simulink model "kay1024_freq_16ch_test"  (R2021b)
settings: Solver=VariableStepAuto  StartTime=0.0  StopTime=10.0  RelTol=1e-3
undefined symbols (not defined in the file): i
libraries: hdlBasic x1194, dspsrcs4 x16, vmcUtilities x1
(part 9 of 14)

== system kay1024_freq_16ch_test/Subsystem/Subsystem16/Subsystem2/CORDIC ATAN/CORDIC Fine Angle PE/CORDIC PE11 ==
  note: X = x - y if y < 0, otherwise
      |    = x + y
      | Y = y + x if y < 0, otherwise
      |    = y - x
      | Z = z - atan(1/2^i) if y < 0, otherwise
      |    = z + atan(1/2^i)
  x : Inport
  y : Inport  Port=2
  z : Inport  Port=3
  AddSub : hdlBasic/AddSub  mode=Addition or Subtraction  use_carryin=off  use_carryout=off  en=off  latency=pipeline  precision=User Defined  arith_type="Signed  (2's comp)"  n_bits=pe_nbits  bin_pt=pe_binpt  quantization=Truncate  overflow=Wrap  use_behavioral_HDL=on  hw_selection=Fabric  pipelined=off  use_rpm=off  XmcBlockStatus=1  maskContainerNames=tabcontainer1  block_type=addsub  block_config=sysgen:Addsub_config
  AddSub1 : hdlBasic/AddSub  mode=Addition or Subtraction  use_carryin=off  use_carryout=off  en=off  latency=pipeline  precision=User Defined  arith_type="Signed  (2's comp)"  n_bits=pe_nbits  bin_pt=pe_binpt  quantization=Truncate  overflow=Wrap  use_behavioral_HDL=on  hw_selection=Fabric  pipelined=off  use_rpm=off  XmcBlockStatus=1  maskContainerNames=tabcontainer1  block_type=addsub  block_config=sysgen:Addsub_config
  AddSub2 : hdlBasic/AddSub  mode=Addition or Subtraction  use_carryin=off  use_carryout=off  en=off  latency=pipeline  precision=User Defined  arith_type="Signed  (2's comp)"  n_bits=pe_nbits  bin_pt=pe_binpt  quantization=Truncate  overflow=Wrap  use_behavioral_HDL=on  hw_selection=Fabric  pipelined=off  use_rpm=off  XmcBlockStatus=1  maskContainerNames=tabcontainer1  block_type=addsub  block_config=sysgen:Addsub_config
  Constant : hdlBasic/Constant  const=epsilon_k  gui_display_data_type=Fixed-point  arith_type=Signed (2's comp)  n_bits=pe_nbits  bin_pt=pe_binpt  preci_type=Single  exp_width=8  frac_width=24  explicit_period=off  period=1  XmcBlockStatus=1  maskContainerNames=tabcontainer1  block_type=constant  block_config=sysgen:Constant_config
  Inverter : hdlBasic/Inverter  en=off  latency=0  XmcBlockStatus=1  maskContainerNames=group2  block_type=inv  block_config=sysgen:Inverter_config
  Shift : hdlBasic/Shift  shift_dir=Right  shift_bits=ii  en=off  latency=0  precision=User Defined  arith_type="Signed  (2's comp)"  n_bits=pe_nbits  bin_pt=pe_binpt  quantization=Truncate  overflow=Wrap  XmcBlockStatus=1  maskContainerNames=group2  block_type=shift  block_config=sysgen:Shift_config
  Shift1 : hdlBasic/Shift  shift_dir=Right  shift_bits=ii  en=off  latency=0  precision=User Defined  arith_type="Signed  (2's comp)"  n_bits=pe_nbits  bin_pt=pe_binpt  quantization=Truncate  overflow=Wrap  XmcBlockStatus=1  maskContainerNames=group2  block_type=shift  block_config=sysgen:Shift_config
  Slice : hdlBasic/Slice  nbits=1  boolean_output=on  mode=Upper Bit Location + Width  bit1=0  base1=MSB of Input  bit0=0  base0=LSB of Input  XmcBlockStatus=1  maskContainerNames=group1  block_type=slice  block_config=sysgen:Slice_config
  X : Outport
  Y : Outport  Port=2
  Z : Outport  Port=3
  wires:
  Slice/1 -> AddSub/3, AddSub2/3, Inverter/1
  Shift1/1 -> AddSub/2
  Shift/1 -> AddSub1/2
  Inverter/1 -> AddSub1/3
  Constant/1 -> AddSub2/2
  AddSub2/1 -> Z/1
  AddSub1/1 -> Y/1
  z/1 -> AddSub2/1
  AddSub/1 -> X/1
  y/1 -> Slice/1, Shift1/1, AddSub1/1
  x/1 -> Shift/1, AddSub/1

== system kay1024_freq_16ch_test/Subsystem/Subsystem16/Subsystem2/CORDIC ATAN/CORDIC Fine Angle PE/CORDIC PE12 ==
  note: X = x - y if y < 0, otherwise
      |    = x + y
      | Y = y + x if y < 0, otherwise
      |    = y - x
      | Z = z - atan(1/2^i) if y < 0, otherwise
      |    = z + atan(1/2^i)
  x : Inport
  y : Inport  Port=2
  z : Inport  Port=3
  AddSub : hdlBasic/AddSub  mode=Addition or Subtraction  use_carryin=off  use_carryout=off  en=off  latency=pipeline  precision=User Defined  arith_type="Signed  (2's comp)"  n_bits=pe_nbits  bin_pt=pe_binpt  quantization=Truncate  overflow=Wrap  use_behavioral_HDL=on  hw_selection=Fabric  pipelined=off  use_rpm=off  XmcBlockStatus=1  maskContainerNames=tabcontainer1  block_type=addsub  block_config=sysgen:Addsub_config
  AddSub1 : hdlBasic/AddSub  mode=Addition or Subtraction  use_carryin=off  use_carryout=off  en=off  latency=pipeline  precision=User Defined  arith_type="Signed  (2's comp)"  n_bits=pe_nbits  bin_pt=pe_binpt  quantization=Truncate  overflow=Wrap  use_behavioral_HDL=on  hw_selection=Fabric  pipelined=off  use_rpm=off  XmcBlockStatus=1  maskContainerNames=tabcontainer1  block_type=addsub  block_config=sysgen:Addsub_config
  AddSub2 : hdlBasic/AddSub  mode=Addition or Subtraction  use_carryin=off  use_carryout=off  en=off  latency=pipeline  precision=User Defined  arith_type="Signed  (2's comp)"  n_bits=pe_nbits  bin_pt=pe_binpt  quantization=Truncate  overflow=Wrap  use_behavioral_HDL=on  hw_selection=Fabric  pipelined=off  use_rpm=off  XmcBlockStatus=1  maskContainerNames=tabcontainer1  block_type=addsub  block_config=sysgen:Addsub_config
  Constant : hdlBasic/Constant  const=epsilon_k  gui_display_data_type=Fixed-point  arith_type=Signed (2's comp)  n_bits=pe_nbits  bin_pt=pe_binpt  preci_type=Single  exp_width=8  frac_width=24  explicit_period=off  period=1  XmcBlockStatus=1  maskContainerNames=tabcontainer1  block_type=constant  block_config=sysgen:Constant_config
  Inverter : hdlBasic/Inverter  en=off  latency=0  XmcBlockStatus=1  maskContainerNames=group2  block_type=inv  block_config=sysgen:Inverter_config
  Shift : hdlBasic/Shift  shift_dir=Right  shift_bits=ii  en=off  latency=0  precision=User Defined  arith_type="Signed  (2's comp)"  n_bits=pe_nbits  bin_pt=pe_binpt  quantization=Truncate  overflow=Wrap  XmcBlockStatus=1  maskContainerNames=group2  block_type=shift  block_config=sysgen:Shift_config
  Shift1 : hdlBasic/Shift  shift_dir=Right  shift_bits=ii  en=off  latency=0  precision=User Defined  arith_type="Signed  (2's comp)"  n_bits=pe_nbits  bin_pt=pe_binpt  quantization=Truncate  overflow=Wrap  XmcBlockStatus=1  maskContainerNames=group2  block_type=shift  block_config=sysgen:Shift_config
  Slice : hdlBasic/Slice  nbits=1  boolean_output=on  mode=Upper Bit Location + Width  bit1=0  base1=MSB of Input  bit0=0  base0=LSB of Input  XmcBlockStatus=1  maskContainerNames=group1  block_type=slice  block_config=sysgen:Slice_config
  X : Outport
  Y : Outport  Port=2
  Z : Outport  Port=3
  wires:
  Slice/1 -> AddSub/3, AddSub2/3, Inverter/1
  Shift1/1 -> AddSub/2
  Shift/1 -> AddSub1/2
  Inverter/1 -> AddSub1/3
  Constant/1 -> AddSub2/2
  AddSub2/1 -> Z/1
  AddSub1/1 -> Y/1
  z/1 -> AddSub2/1
  AddSub/1 -> X/1
  y/1 -> Slice/1, Shift1/1, AddSub1/1
  x/1 -> Shift/1, AddSub/1

== system kay1024_freq_16ch_test/Subsystem/Subsystem16/Subsystem2/CORDIC ATAN/CORDIC Fine Angle PE/CORDIC PE13 ==
  note: X = x - y if y < 0, otherwise
      |    = x + y
      | Y = y + x if y < 0, otherwise
      |    = y - x
      | Z = z - atan(1/2^i) if y < 0, otherwise
      |    = z + atan(1/2^i)
  x : Inport
  y : Inport  Port=2
  z : Inport  Port=3
  AddSub : hdlBasic/AddSub  mode=Addition or Subtraction  use_carryin=off  use_carryout=off  en=off  latency=pipeline  precision=User Defined  arith_type="Signed  (2's comp)"  n_bits=pe_nbits  bin_pt=pe_binpt  quantization=Truncate  overflow=Wrap  use_behavioral_HDL=on  hw_selection=Fabric  pipelined=off  use_rpm=off  XmcBlockStatus=1  maskContainerNames=tabcontainer1  block_type=addsub  block_config=sysgen:Addsub_config
  AddSub1 : hdlBasic/AddSub  mode=Addition or Subtraction  use_carryin=off  use_carryout=off  en=off  latency=pipeline  precision=User Defined  arith_type="Signed  (2's comp)"  n_bits=pe_nbits  bin_pt=pe_binpt  quantization=Truncate  overflow=Wrap  use_behavioral_HDL=on  hw_selection=Fabric  pipelined=off  use_rpm=off  XmcBlockStatus=1  maskContainerNames=tabcontainer1  block_type=addsub  block_config=sysgen:Addsub_config
  AddSub2 : hdlBasic/AddSub  mode=Addition or Subtraction  use_carryin=off  use_carryout=off  en=off  latency=pipeline  precision=User Defined  arith_type="Signed  (2's comp)"  n_bits=pe_nbits  bin_pt=pe_binpt  quantization=Truncate  overflow=Wrap  use_behavioral_HDL=on  hw_selection=Fabric  pipelined=off  use_rpm=off  XmcBlockStatus=1  maskContainerNames=tabcontainer1  block_type=addsub  block_config=sysgen:Addsub_config
  Constant : hdlBasic/Constant  const=epsilon_k  gui_display_data_type=Fixed-point  arith_type=Signed (2's comp)  n_bits=pe_nbits  bin_pt=pe_binpt  preci_type=Single  exp_width=8  frac_width=24  explicit_period=off  period=1  XmcBlockStatus=1  maskContainerNames=tabcontainer1  block_type=constant  block_config=sysgen:Constant_config
  Inverter : hdlBasic/Inverter  en=off  latency=0  XmcBlockStatus=1  maskContainerNames=group2  block_type=inv  block_config=sysgen:Inverter_config
  Shift : hdlBasic/Shift  shift_dir=Right  shift_bits=ii  en=off  latency=0  precision=User Defined  arith_type="Signed  (2's comp)"  n_bits=pe_nbits  bin_pt=pe_binpt  quantization=Truncate  overflow=Wrap  XmcBlockStatus=1  maskContainerNames=group2  block_type=shift  block_config=sysgen:Shift_config
  Shift1 : hdlBasic/Shift  shift_dir=Right  shift_bits=ii  en=off  latency=0  precision=User Defined  arith_type="Signed  (2's comp)"  n_bits=pe_nbits  bin_pt=pe_binpt  quantization=Truncate  overflow=Wrap  XmcBlockStatus=1  maskContainerNames=group2  block_type=shift  block_config=sysgen:Shift_config
  Slice : hdlBasic/Slice  nbits=1  boolean_output=on  mode=Upper Bit Location + Width  bit1=0  base1=MSB of Input  bit0=0  base0=LSB of Input  XmcBlockStatus=1  maskContainerNames=group1  block_type=slice  block_config=sysgen:Slice_config
  X : Outport
  Y : Outport  Port=2
  Z : Outport  Port=3
  wires:
  Slice/1 -> AddSub/3, AddSub2/3, Inverter/1
  Shift1/1 -> AddSub/2
  Shift/1 -> AddSub1/2
  Inverter/1 -> AddSub1/3
  Constant/1 -> AddSub2/2
  AddSub2/1 -> Z/1
  AddSub1/1 -> Y/1
  z/1 -> AddSub2/1
  AddSub/1 -> X/1
  y/1 -> Slice/1, Shift1/1, AddSub1/1
  x/1 -> Shift/1, AddSub/1

== system kay1024_freq_16ch_test/Subsystem/Subsystem16/Subsystem2/CORDIC ATAN/CORDIC Fine Angle PE/CORDIC PE14 ==
  note: X = x - y if y < 0, otherwise
      |    = x + y
      | Y = y + x if y < 0, otherwise
      |    = y - x
      | Z = z - atan(1/2^i) if y < 0, otherwise
      |    = z + atan(1/2^i)
  x : Inport
  y : Inport  Port=2
  z : Inport  Port=3
  AddSub : hdlBasic/AddSub  mode=Addition or Subtraction  use_carryin=off  use_carryout=off  en=off  latency=pipeline  precision=User Defined  arith_type="Signed  (2's comp)"  n_bits=pe_nbits  bin_pt=pe_binpt  quantization=Truncate  overflow=Wrap  use_behavioral_HDL=on  hw_selection=Fabric  pipelined=off  use_rpm=off  XmcBlockStatus=1  maskContainerNames=tabcontainer1  block_type=addsub  block_config=sysgen:Addsub_config
  AddSub1 : hdlBasic/AddSub  mode=Addition or Subtraction  use_carryin=off  use_carryout=off  en=off  latency=pipeline  precision=User Defined  arith_type="Signed  (2's comp)"  n_bits=pe_nbits  bin_pt=pe_binpt  quantization=Truncate  overflow=Wrap  use_behavioral_HDL=on  hw_selection=Fabric  pipelined=off  use_rpm=off  XmcBlockStatus=1  maskContainerNames=tabcontainer1  block_type=addsub  block_config=sysgen:Addsub_config
  AddSub2 : hdlBasic/AddSub  mode=Addition or Subtraction  use_carryin=off  use_carryout=off  en=off  latency=pipeline  precision=User Defined  arith_type="Signed  (2's comp)"  n_bits=pe_nbits  bin_pt=pe_binpt  quantization=Truncate  overflow=Wrap  use_behavioral_HDL=on  hw_selection=Fabric  pipelined=off  use_rpm=off  XmcBlockStatus=1  maskContainerNames=tabcontainer1  block_type=addsub  block_config=sysgen:Addsub_config
  Constant : hdlBasic/Constant  const=epsilon_k  gui_display_data_type=Fixed-point  arith_type=Signed (2's comp)  n_bits=pe_nbits  bin_pt=pe_binpt  preci_type=Single  exp_width=8  frac_width=24  explicit_period=off  period=1  XmcBlockStatus=1  maskContainerNames=tabcontainer1  block_type=constant  block_config=sysgen:Constant_config
  Inverter : hdlBasic/Inverter  en=off  latency=0  XmcBlockStatus=1  maskContainerNames=group2  block_type=inv  block_config=sysgen:Inverter_config
  Shift : hdlBasic/Shift  shift_dir=Right  shift_bits=ii  en=off  latency=0  precision=User Defined  arith_type="Signed  (2's comp)"  n_bits=pe_nbits  bin_pt=pe_binpt  quantization=Truncate  overflow=Wrap  XmcBlockStatus=1  maskContainerNames=group2  block_type=shift  block_config=sysgen:Shift_config
  Shift1 : hdlBasic/Shift  shift_dir=Right  shift_bits=ii  en=off  latency=0  precision=User Defined  arith_type="Signed  (2's comp)"  n_bits=pe_nbits  bin_pt=pe_binpt  quantization=Truncate  overflow=Wrap  XmcBlockStatus=1  maskContainerNames=group2  block_type=shift  block_config=sysgen:Shift_config
  Slice : hdlBasic/Slice  nbits=1  boolean_output=on  mode=Upper Bit Location + Width  bit1=0  base1=MSB of Input  bit0=0  base0=LSB of Input  XmcBlockStatus=1  maskContainerNames=group1  block_type=slice  block_config=sysgen:Slice_config
  X : Outport
  Y : Outport  Port=2
  Z : Outport  Port=3
  wires:
  Slice/1 -> AddSub/3, AddSub2/3, Inverter/1
  Shift1/1 -> AddSub/2
  Shift/1 -> AddSub1/2
  Inverter/1 -> AddSub1/3
  Constant/1 -> AddSub2/2
  AddSub2/1 -> Z/1
  AddSub1/1 -> Y/1
  z/1 -> AddSub2/1
  AddSub/1 -> X/1
  y/1 -> Slice/1, Shift1/1, AddSub1/1
  x/1 -> Shift/1, AddSub/1

== system kay1024_freq_16ch_test/Subsystem/Subsystem16/Subsystem2/CORDIC ATAN/CORDIC Fine Angle PE/CORDIC PE15 ==
  note: X = x - y if y < 0, otherwise
      |    = x + y
      | Y = y + x if y < 0, otherwise
      |    = y - x
      | Z = z - atan(1/2^i) if y < 0, otherwise
      |    = z + atan(1/2^i)
  x : Inport
  y : Inport  Port=2
  z : Inport  Port=3
  AddSub : hdlBasic/AddSub  mode=Addition or Subtraction  use_carryin=off  use_carryout=off  en=off  latency=pipeline  precision=User Defined  arith_type="Signed  (2's comp)"  n_bits=pe_nbits  bin_pt=pe_binpt  quantization=Truncate  overflow=Wrap  use_behavioral_HDL=on  hw_selection=Fabric  pipelined=off  use_rpm=off  XmcBlockStatus=1  maskContainerNames=tabcontainer1  block_type=addsub  block_config=sysgen:Addsub_config
  AddSub1 : hdlBasic/AddSub  mode=Addition or Subtraction  use_carryin=off  use_carryout=off  en=off  latency=pipeline  precision=User Defined  arith_type="Signed  (2's comp)"  n_bits=pe_nbits  bin_pt=pe_binpt  quantization=Truncate  overflow=Wrap  use_behavioral_HDL=on  hw_selection=Fabric  pipelined=off  use_rpm=off  XmcBlockStatus=1  maskContainerNames=tabcontainer1  block_type=addsub  block_config=sysgen:Addsub_config
  AddSub2 : hdlBasic/AddSub  mode=Addition or Subtraction  use_carryin=off  use_carryout=off  en=off  latency=pipeline  precision=User Defined  arith_type="Signed  (2's comp)"  n_bits=pe_nbits  bin_pt=pe_binpt  quantization=Truncate  overflow=Wrap  use_behavioral_HDL=on  hw_selection=Fabric  pipelined=off  use_rpm=off  XmcBlockStatus=1  maskContainerNames=tabcontainer1  block_type=addsub  block_config=sysgen:Addsub_config
  Constant : hdlBasic/Constant  const=epsilon_k  gui_display_data_type=Fixed-point  arith_type=Signed (2's comp)  n_bits=pe_nbits  bin_pt=pe_binpt  preci_type=Single  exp_width=8  frac_width=24  explicit_period=off  period=1  XmcBlockStatus=1  maskContainerNames=tabcontainer1  block_type=constant  block_config=sysgen:Constant_config
  Inverter : hdlBasic/Inverter  en=off  latency=0  XmcBlockStatus=1  maskContainerNames=group2  block_type=inv  block_config=sysgen:Inverter_config
  Shift : hdlBasic/Shift  shift_dir=Right  shift_bits=ii  en=off  latency=0  precision=User Defined  arith_type="Signed  (2's comp)"  n_bits=pe_nbits  bin_pt=pe_binpt  quantization=Truncate  overflow=Wrap  XmcBlockStatus=1  maskContainerNames=group2  block_type=shift  block_config=sysgen:Shift_config
  Shift1 : hdlBasic/Shift  shift_dir=Right  shift_bits=ii  en=off  latency=0  precision=User Defined  arith_type="Signed  (2's comp)"  n_bits=pe_nbits  bin_pt=pe_binpt  quantization=Truncate  overflow=Wrap  XmcBlockStatus=1  maskContainerNames=group2  block_type=shift  block_config=sysgen:Shift_config
  Slice : hdlBasic/Slice  nbits=1  boolean_output=on  mode=Upper Bit Location + Width  bit1=0  base1=MSB of Input  bit0=0  base0=LSB of Input  XmcBlockStatus=1  maskContainerNames=group1  block_type=slice  block_config=sysgen:Slice_config
  X : Outport
  Y : Outport  Port=2
  Z : Outport  Port=3
  wires:
  Slice/1 -> AddSub/3, AddSub2/3, Inverter/1
  Shift1/1 -> AddSub/2
  Shift/1 -> AddSub1/2
  Inverter/1 -> AddSub1/3
  Constant/1 -> AddSub2/2
  AddSub2/1 -> Z/1
  AddSub1/1 -> Y/1
  z/1 -> AddSub2/1
  AddSub/1 -> X/1
  y/1 -> Slice/1, Shift1/1, AddSub1/1
  x/1 -> Shift/1, AddSub/1

== system kay1024_freq_16ch_test/Subsystem/Subsystem16/Subsystem2/CORDIC ATAN/CORDIC Fine Angle PE/CORDIC PE2 ==
  note: X = x - y if y < 0, otherwise
      |    = x + y
      | Y = y + x if y < 0, otherwise
      |    = y - x
      | Z = z - atan(1/2^i) if y < 0, otherwise
      |    = z + atan(1/2^i)
  x : Inport
  y : Inport  Port=2
  z : Inport  Port=3
  AddSub : hdlBasic/AddSub  mode=Addition or Subtraction  use_carryin=off  use_carryout=off  en=off  latency=pipeline  precision=User Defined  arith_type="Signed  (2's comp)"  n_bits=pe_nbits  bin_pt=pe_binpt  quantization=Truncate  overflow=Wrap  use_behavioral_HDL=on  hw_selection=Fabric  pipelined=off  use_rpm=off  XmcBlockStatus=1  maskContainerNames=tabcontainer1  block_type=addsub  block_config=sysgen:Addsub_config
  AddSub1 : hdlBasic/AddSub  mode=Addition or Subtraction  use_carryin=off  use_carryout=off  en=off  latency=pipeline  precision=User Defined  arith_type="Signed  (2's comp)"  n_bits=pe_nbits  bin_pt=pe_binpt  quantization=Truncate  overflow=Wrap  use_behavioral_HDL=on  hw_selection=Fabric  pipelined=off  use_rpm=off  XmcBlockStatus=1  maskContainerNames=tabcontainer1  block_type=addsub  block_config=sysgen:Addsub_config
  AddSub2 : hdlBasic/AddSub  mode=Addition or Subtraction  use_carryin=off  use_carryout=off  en=off  latency=pipeline  precision=User Defined  arith_type="Signed  (2's comp)"  n_bits=pe_nbits  bin_pt=pe_binpt  quantization=Truncate  overflow=Wrap  use_behavioral_HDL=on  hw_selection=Fabric  pipelined=off  use_rpm=off  XmcBlockStatus=1  maskContainerNames=tabcontainer1  block_type=addsub  block_config=sysgen:Addsub_config
  Constant : hdlBasic/Constant  const=epsilon_k  gui_display_data_type=Fixed-point  arith_type=Signed (2's comp)  n_bits=pe_nbits  bin_pt=pe_binpt  preci_type=Single  exp_width=8  frac_width=24  explicit_period=off  period=1  XmcBlockStatus=1  maskContainerNames=tabcontainer1  block_type=constant  block_config=sysgen:Constant_config
  Inverter : hdlBasic/Inverter  en=off  latency=0  XmcBlockStatus=1  maskContainerNames=group2  block_type=inv  block_config=sysgen:Inverter_config
  Shift : hdlBasic/Shift  shift_dir=Right  shift_bits=ii  en=off  latency=0  precision=User Defined  arith_type="Signed  (2's comp)"  n_bits=pe_nbits  bin_pt=pe_binpt  quantization=Truncate  overflow=Wrap  XmcBlockStatus=1  maskContainerNames=group2  block_type=shift  block_config=sysgen:Shift_config
  Shift1 : hdlBasic/Shift  shift_dir=Right  shift_bits=ii  en=off  latency=0  precision=User Defined  arith_type="Signed  (2's comp)"  n_bits=pe_nbits  bin_pt=pe_binpt  quantization=Truncate  overflow=Wrap  XmcBlockStatus=1  maskContainerNames=group2  block_type=shift  block_config=sysgen:Shift_config
  Slice : hdlBasic/Slice  nbits=1  boolean_output=on  mode=Upper Bit Location + Width  bit1=0  base1=MSB of Input  bit0=0  base0=LSB of Input  XmcBlockStatus=1  maskContainerNames=group1  block_type=slice  block_config=sysgen:Slice_config
  X : Outport
  Y : Outport  Port=2
  Z : Outport  Port=3
  wires:
  Slice/1 -> AddSub/3, AddSub2/3, Inverter/1
  Shift1/1 -> AddSub/2
  Shift/1 -> AddSub1/2
  Inverter/1 -> AddSub1/3
  Constant/1 -> AddSub2/2
  AddSub2/1 -> Z/1
  AddSub1/1 -> Y/1
  z/1 -> AddSub2/1
  AddSub/1 -> X/1
  y/1 -> Slice/1, Shift1/1, AddSub1/1
  x/1 -> Shift/1, AddSub/1

== system kay1024_freq_16ch_test/Subsystem/Subsystem16/Subsystem2/CORDIC ATAN/CORDIC Fine Angle PE/CORDIC PE3 ==
  note: X = x - y if y < 0, otherwise
      |    = x + y
      | Y = y + x if y < 0, otherwise
      |    = y - x
      | Z = z - atan(1/2^i) if y < 0, otherwise
      |    = z + atan(1/2^i)
  x : Inport
  y : Inport  Port=2
  z : Inport  Port=3
  AddSub : hdlBasic/AddSub  mode=Addition or Subtraction  use_carryin=off  use_carryout=off  en=off  latency=pipeline  precision=User Defined  arith_type="Signed  (2's comp)"  n_bits=pe_nbits  bin_pt=pe_binpt  quantization=Truncate  overflow=Wrap  use_behavioral_HDL=on  hw_selection=Fabric  pipelined=off  use_rpm=off  XmcBlockStatus=1  maskContainerNames=tabcontainer1  block_type=addsub  block_config=sysgen:Addsub_config
  AddSub1 : hdlBasic/AddSub  mode=Addition or Subtraction  use_carryin=off  use_carryout=off  en=off  latency=pipeline  precision=User Defined  arith_type="Signed  (2's comp)"  n_bits=pe_nbits  bin_pt=pe_binpt  quantization=Truncate  overflow=Wrap  use_behavioral_HDL=on  hw_selection=Fabric  pipelined=off  use_rpm=off  XmcBlockStatus=1  maskContainerNames=tabcontainer1  block_type=addsub  block_config=sysgen:Addsub_config
  AddSub2 : hdlBasic/AddSub  mode=Addition or Subtraction  use_carryin=off  use_carryout=off  en=off  latency=pipeline  precision=User Defined  arith_type="Signed  (2's comp)"  n_bits=pe_nbits  bin_pt=pe_binpt  quantization=Truncate  overflow=Wrap  use_behavioral_HDL=on  hw_selection=Fabric  pipelined=off  use_rpm=off  XmcBlockStatus=1  maskContainerNames=tabcontainer1  block_type=addsub  block_config=sysgen:Addsub_config
  Constant : hdlBasic/Constant  const=epsilon_k  gui_display_data_type=Fixed-point  arith_type=Signed (2's comp)  n_bits=pe_nbits  bin_pt=pe_binpt  preci_type=Single  exp_width=8  frac_width=24  explicit_period=off  period=1  XmcBlockStatus=1  maskContainerNames=tabcontainer1  block_type=constant  block_config=sysgen:Constant_config
  Inverter : hdlBasic/Inverter  en=off  latency=0  XmcBlockStatus=1  maskContainerNames=group2  block_type=inv  block_config=sysgen:Inverter_config
  Shift : hdlBasic/Shift  shift_dir=Right  shift_bits=ii  en=off  latency=0  precision=User Defined  arith_type="Signed  (2's comp)"  n_bits=pe_nbits  bin_pt=pe_binpt  quantization=Truncate  overflow=Wrap  XmcBlockStatus=1  maskContainerNames=group2  block_type=shift  block_config=sysgen:Shift_config
  Shift1 : hdlBasic/Shift  shift_dir=Right  shift_bits=ii  en=off  latency=0  precision=User Defined  arith_type="Signed  (2's comp)"  n_bits=pe_nbits  bin_pt=pe_binpt  quantization=Truncate  overflow=Wrap  XmcBlockStatus=1  maskContainerNames=group2  block_type=shift  block_config=sysgen:Shift_config
  Slice : hdlBasic/Slice  nbits=1  boolean_output=on  mode=Upper Bit Location + Width  bit1=0  base1=MSB of Input  bit0=0  base0=LSB of Input  XmcBlockStatus=1  maskContainerNames=group1  block_type=slice  block_config=sysgen:Slice_config
  X : Outport
  Y : Outport  Port=2
  Z : Outport  Port=3
  wires:
  Slice/1 -> AddSub/3, AddSub2/3, Inverter/1
  Shift1/1 -> AddSub/2
  Shift/1 -> AddSub1/2
  Inverter/1 -> AddSub1/3
  Constant/1 -> AddSub2/2
  AddSub2/1 -> Z/1
  AddSub1/1 -> Y/1
  z/1 -> AddSub2/1
  AddSub/1 -> X/1
  y/1 -> Slice/1, Shift1/1, AddSub1/1
  x/1 -> Shift/1, AddSub/1

== system kay1024_freq_16ch_test/Subsystem/Subsystem16/Subsystem2/CORDIC ATAN/CORDIC Fine Angle PE/CORDIC PE4 ==
  note: X = x - y if y < 0, otherwise
      |    = x + y
      | Y = y + x if y < 0, otherwise
      |    = y - x
      | Z = z - atan(1/2^i) if y < 0, otherwise
      |    = z + atan(1/2^i)
  x : Inport
  y : Inport  Port=2
  z : Inport  Port=3
  AddSub : hdlBasic/AddSub  mode=Addition or Subtraction  use_carryin=off  use_carryout=off  en=off  latency=pipeline  precision=User Defined  arith_type="Signed  (2's comp)"  n_bits=pe_nbits  bin_pt=pe_binpt  quantization=Truncate  overflow=Wrap  use_behavioral_HDL=on  hw_selection=Fabric  pipelined=off  use_rpm=off  XmcBlockStatus=1  maskContainerNames=tabcontainer1  block_type=addsub  block_config=sysgen:Addsub_config
  AddSub1 : hdlBasic/AddSub  mode=Addition or Subtraction  use_carryin=off  use_carryout=off  en=off  latency=pipeline  precision=User Defined  arith_type="Signed  (2's comp)"  n_bits=pe_nbits  bin_pt=pe_binpt  quantization=Truncate  overflow=Wrap  use_behavioral_HDL=on  hw_selection=Fabric  pipelined=off  use_rpm=off  XmcBlockStatus=1  maskContainerNames=tabcontainer1  block_type=addsub  block_config=sysgen:Addsub_config
  AddSub2 : hdlBasic/AddSub  mode=Addition or Subtraction  use_carryin=off  use_carryout=off  en=off  latency=pipeline  precision=User Defined  arith_type="Signed  (2's comp)"  n_bits=pe_nbits  bin_pt=pe_binpt  quantization=Truncate  overflow=Wrap  use_behavioral_HDL=on  hw_selection=Fabric  pipelined=off  use_rpm=off  XmcBlockStatus=1  maskContainerNames=tabcontainer1  block_type=addsub  block_config=sysgen:Addsub_config
  Constant : hdlBasic/Constant  const=epsilon_k  gui_display_data_type=Fixed-point  arith_type=Signed (2's comp)  n_bits=pe_nbits  bin_pt=pe_binpt  preci_type=Single  exp_width=8  frac_width=24  explicit_period=off  period=1  XmcBlockStatus=1  maskContainerNames=tabcontainer1  block_type=constant  block_config=sysgen:Constant_config
  Inverter : hdlBasic/Inverter  en=off  latency=0  XmcBlockStatus=1  maskContainerNames=group2  block_type=inv  block_config=sysgen:Inverter_config
  Shift : hdlBasic/Shift  shift_dir=Right  shift_bits=ii  en=off  latency=0  precision=User Defined  arith_type="Signed  (2's comp)"  n_bits=pe_nbits  bin_pt=pe_binpt  quantization=Truncate  overflow=Wrap  XmcBlockStatus=1  maskContainerNames=group2  block_type=shift  block_config=sysgen:Shift_config
  Shift1 : hdlBasic/Shift  shift_dir=Right  shift_bits=ii  en=off  latency=0  precision=User Defined  arith_type="Signed  (2's comp)"  n_bits=pe_nbits  bin_pt=pe_binpt  quantization=Truncate  overflow=Wrap  XmcBlockStatus=1  maskContainerNames=group2  block_type=shift  block_config=sysgen:Shift_config
  Slice : hdlBasic/Slice  nbits=1  boolean_output=on  mode=Upper Bit Location + Width  bit1=0  base1=MSB of Input  bit0=0  base0=LSB of Input  XmcBlockStatus=1  maskContainerNames=group1  block_type=slice  block_config=sysgen:Slice_config
  X : Outport
  Y : Outport  Port=2
  Z : Outport  Port=3
  wires:
  Slice/1 -> AddSub/3, AddSub2/3, Inverter/1
  Shift1/1 -> AddSub/2
  Shift/1 -> AddSub1/2
  Inverter/1 -> AddSub1/3
  Constant/1 -> AddSub2/2
  AddSub2/1 -> Z/1
  AddSub1/1 -> Y/1
  z/1 -> AddSub2/1
  AddSub/1 -> X/1
  y/1 -> Slice/1, Shift1/1, AddSub1/1
  x/1 -> Shift/1, AddSub/1

== system kay1024_freq_16ch_test/Subsystem/Subsystem16/Subsystem2/CORDIC ATAN/CORDIC Fine Angle PE/CORDIC PE5 ==
  note: X = x - y if y < 0, otherwise
      |    = x + y
      | Y = y + x if y < 0, otherwise
      |    = y - x
      | Z = z - atan(1/2^i) if y < 0, otherwise
      |    = z + atan(1/2^i)
  x : Inport
  y : Inport  Port=2
  z : Inport  Port=3
  AddSub : hdlBasic/AddSub  mode=Addition or Subtraction  use_carryin=off  use_carryout=off  en=off  latency=pipeline  precision=User Defined  arith_type="Signed  (2's comp)"  n_bits=pe_nbits  bin_pt=pe_binpt  quantization=Truncate  overflow=Wrap  use_behavioral_HDL=on  hw_selection=Fabric  pipelined=off  use_rpm=off  XmcBlockStatus=1  maskContainerNames=tabcontainer1  block_type=addsub  block_config=sysgen:Addsub_config
  AddSub1 : hdlBasic/AddSub  mode=Addition or Subtraction  use_carryin=off  use_carryout=off  en=off  latency=pipeline  precision=User Defined  arith_type="Signed  (2's comp)"  n_bits=pe_nbits  bin_pt=pe_binpt  quantization=Truncate  overflow=Wrap  use_behavioral_HDL=on  hw_selection=Fabric  pipelined=off  use_rpm=off  XmcBlockStatus=1  maskContainerNames=tabcontainer1  block_type=addsub  block_config=sysgen:Addsub_config
  AddSub2 : hdlBasic/AddSub  mode=Addition or Subtraction  use_carryin=off  use_carryout=off  en=off  latency=pipeline  precision=User Defined  arith_type="Signed  (2's comp)"  n_bits=pe_nbits  bin_pt=pe_binpt  quantization=Truncate  overflow=Wrap  use_behavioral_HDL=on  hw_selection=Fabric  pipelined=off  use_rpm=off  XmcBlockStatus=1  maskContainerNames=tabcontainer1  block_type=addsub  block_config=sysgen:Addsub_config
  Constant : hdlBasic/Constant  const=epsilon_k  gui_display_data_type=Fixed-point  arith_type=Signed (2's comp)  n_bits=pe_nbits  bin_pt=pe_binpt  preci_type=Single  exp_width=8  frac_width=24  explicit_period=off  period=1  XmcBlockStatus=1  maskContainerNames=tabcontainer1  block_type=constant  block_config=sysgen:Constant_config
  Inverter : hdlBasic/Inverter  en=off  latency=0  XmcBlockStatus=1  maskContainerNames=group2  block_type=inv  block_config=sysgen:Inverter_config
  Shift : hdlBasic/Shift  shift_dir=Right  shift_bits=ii  en=off  latency=0  precision=User Defined  arith_type="Signed  (2's comp)"  n_bits=pe_nbits  bin_pt=pe_binpt  quantization=Truncate  overflow=Wrap  XmcBlockStatus=1  maskContainerNames=group2  block_type=shift  block_config=sysgen:Shift_config
  Shift1 : hdlBasic/Shift  shift_dir=Right  shift_bits=ii  en=off  latency=0  precision=User Defined  arith_type="Signed  (2's comp)"  n_bits=pe_nbits  bin_pt=pe_binpt  quantization=Truncate  overflow=Wrap  XmcBlockStatus=1  maskContainerNames=group2  block_type=shift  block_config=sysgen:Shift_config
  Slice : hdlBasic/Slice  nbits=1  boolean_output=on  mode=Upper Bit Location + Width  bit1=0  base1=MSB of Input  bit0=0  base0=LSB of Input  XmcBlockStatus=1  maskContainerNames=group1  block_type=slice  block_config=sysgen:Slice_config
  X : Outport
  Y : Outport  Port=2
  Z : Outport  Port=3
  wires:
  Slice/1 -> AddSub/3, AddSub2/3, Inverter/1
  Shift1/1 -> AddSub/2
  Shift/1 -> AddSub1/2
  Inverter/1 -> AddSub1/3
  Constant/1 -> AddSub2/2
  AddSub2/1 -> Z/1
  AddSub1/1 -> Y/1
  z/1 -> AddSub2/1
  AddSub/1 -> X/1
  y/1 -> Slice/1, Shift1/1, AddSub1/1
  x/1 -> Shift/1, AddSub/1

== system kay1024_freq_16ch_test/Subsystem/Subsystem16/Subsystem2/CORDIC ATAN/CORDIC Fine Angle PE/CORDIC PE6 ==
  note: X = x - y if y < 0, otherwise
      |    = x + y
      | Y = y + x if y < 0, otherwise
      |    = y - x
      | Z = z - atan(1/2^i) if y < 0, otherwise
      |    = z + atan(1/2^i)
  x : Inport
  y : Inport  Port=2
  z : Inport  Port=3
  AddSub : hdlBasic/AddSub  mode=Addition or Subtraction  use_carryin=off  use_carryout=off  en=off  latency=pipeline  precision=User Defined  arith_type="Signed  (2's comp)"  n_bits=pe_nbits  bin_pt=pe_binpt  quantization=Truncate  overflow=Wrap  use_behavioral_HDL=on  hw_selection=Fabric  pipelined=off  use_rpm=off  XmcBlockStatus=1  maskContainerNames=tabcontainer1  block_type=addsub  block_config=sysgen:Addsub_config
  AddSub1 : hdlBasic/AddSub  mode=Addition or Subtraction  use_carryin=off  use_carryout=off  en=off  latency=pipeline  precision=User Defined  arith_type="Signed  (2's comp)"  n_bits=pe_nbits  bin_pt=pe_binpt  quantization=Truncate  overflow=Wrap  use_behavioral_HDL=on  hw_selection=Fabric  pipelined=off  use_rpm=off  XmcBlockStatus=1  maskContainerNames=tabcontainer1  block_type=addsub  block_config=sysgen:Addsub_config
  AddSub2 : hdlBasic/AddSub  mode=Addition or Subtraction  use_carryin=off  use_carryout=off  en=off  latency=pipeline  precision=User Defined  arith_type="Signed  (2's comp)"  n_bits=pe_nbits  bin_pt=pe_binpt  quantization=Truncate  overflow=Wrap  use_behavioral_HDL=on  hw_selection=Fabric  pipelined=off  use_rpm=off  XmcBlockStatus=1  maskContainerNames=tabcontainer1  block_type=addsub  block_config=sysgen:Addsub_config
  Constant : hdlBasic/Constant  const=epsilon_k  gui_display_data_type=Fixed-point  arith_type=Signed (2's comp)  n_bits=pe_nbits  bin_pt=pe_binpt  preci_type=Single  exp_width=8  frac_width=24  explicit_period=off  period=1  XmcBlockStatus=1  maskContainerNames=tabcontainer1  block_type=constant  block_config=sysgen:Constant_config
  Inverter : hdlBasic/Inverter  en=off  latency=0  XmcBlockStatus=1  maskContainerNames=group2  block_type=inv  block_config=sysgen:Inverter_config
  Shift : hdlBasic/Shift  shift_dir=Right  shift_bits=ii  en=off  latency=0  precision=User Defined  arith_type="Signed  (2's comp)"  n_bits=pe_nbits  bin_pt=pe_binpt  quantization=Truncate  overflow=Wrap  XmcBlockStatus=1  maskContainerNames=group2  block_type=shift  block_config=sysgen:Shift_config
  Shift1 : hdlBasic/Shift  shift_dir=Right  shift_bits=ii  en=off  latency=0  precision=User Defined  arith_type="Signed  (2's comp)"  n_bits=pe_nbits  bin_pt=pe_binpt  quantization=Truncate  overflow=Wrap  XmcBlockStatus=1  maskContainerNames=group2  block_type=shift  block_config=sysgen:Shift_config
  Slice : hdlBasic/Slice  nbits=1  boolean_output=on  mode=Upper Bit Location + Width  bit1=0  base1=MSB of Input  bit0=0  base0=LSB of Input  XmcBlockStatus=1  maskContainerNames=group1  block_type=slice  block_config=sysgen:Slice_config
  X : Outport
  Y : Outport  Port=2
  Z : Outport  Port=3
  wires:
  Slice/1 -> AddSub/3, AddSub2/3, Inverter/1
  Shift1/1 -> AddSub/2
  Shift/1 -> AddSub1/2
  Inverter/1 -> AddSub1/3
  Constant/1 -> AddSub2/2
  AddSub2/1 -> Z/1
  AddSub1/1 -> Y/1
  z/1 -> AddSub2/1
  AddSub/1 -> X/1
  y/1 -> Slice/1, Shift1/1, AddSub1/1
  x/1 -> Shift/1, AddSub/1

== system kay1024_freq_16ch_test/Subsystem/Subsystem16/Subsystem2/CORDIC ATAN/CORDIC Fine Angle PE/CORDIC PE7 ==
  note: X = x - y if y < 0, otherwise
      |    = x + y
      | Y = y + x if y < 0, otherwise
      |    = y - x
      | Z = z - atan(1/2^i) if y < 0, otherwise
      |    = z + atan(1/2^i)
  x : Inport
  y : Inport  Port=2
  z : Inport  Port=3
  AddSub : hdlBasic/AddSub  mode=Addition or Subtraction  use_carryin=off  use_carryout=off  en=off  latency=pipeline  precision=User Defined  arith_type="Signed  (2's comp)"  n_bits=pe_nbits  bin_pt=pe_binpt  quantization=Truncate  overflow=Wrap  use_behavioral_HDL=on  hw_selection=Fabric  pipelined=off  use_rpm=off  XmcBlockStatus=1  maskContainerNames=tabcontainer1  block_type=addsub  block_config=sysgen:Addsub_config
  AddSub1 : hdlBasic/AddSub  mode=Addition or Subtraction  use_carryin=off  use_carryout=off  en=off  latency=pipeline  precision=User Defined  arith_type="Signed  (2's comp)"  n_bits=pe_nbits  bin_pt=pe_binpt  quantization=Truncate  overflow=Wrap  use_behavioral_HDL=on  hw_selection=Fabric  pipelined=off  use_rpm=off  XmcBlockStatus=1  maskContainerNames=tabcontainer1  block_type=addsub  block_config=sysgen:Addsub_config
  AddSub2 : hdlBasic/AddSub  mode=Addition or Subtraction  use_carryin=off  use_carryout=off  en=off  latency=pipeline  precision=User Defined  arith_type="Signed  (2's comp)"  n_bits=pe_nbits  bin_pt=pe_binpt  quantization=Truncate  overflow=Wrap  use_behavioral_HDL=on  hw_selection=Fabric  pipelined=off  use_rpm=off  XmcBlockStatus=1  maskContainerNames=tabcontainer1  block_type=addsub  block_config=sysgen:Addsub_config
  Constant : hdlBasic/Constant  const=epsilon_k  gui_display_data_type=Fixed-point  arith_type=Signed (2's comp)  n_bits=pe_nbits  bin_pt=pe_binpt  preci_type=Single  exp_width=8  frac_width=24  explicit_period=off  period=1  XmcBlockStatus=1  maskContainerNames=tabcontainer1  block_type=constant  block_config=sysgen:Constant_config
  Inverter : hdlBasic/Inverter  en=off  latency=0  XmcBlockStatus=1  maskContainerNames=group2  block_type=inv  block_config=sysgen:Inverter_config
  Shift : hdlBasic/Shift  shift_dir=Right  shift_bits=ii  en=off  latency=0  precision=User Defined  arith_type="Signed  (2's comp)"  n_bits=pe_nbits  bin_pt=pe_binpt  quantization=Truncate  overflow=Wrap  XmcBlockStatus=1  maskContainerNames=group2  block_type=shift  block_config=sysgen:Shift_config
  Shift1 : hdlBasic/Shift  shift_dir=Right  shift_bits=ii  en=off  latency=0  precision=User Defined  arith_type="Signed  (2's comp)"  n_bits=pe_nbits  bin_pt=pe_binpt  quantization=Truncate  overflow=Wrap  XmcBlockStatus=1  maskContainerNames=group2  block_type=shift  block_config=sysgen:Shift_config
  Slice : hdlBasic/Slice  nbits=1  boolean_output=on  mode=Upper Bit Location + Width  bit1=0  base1=MSB of Input  bit0=0  base0=LSB of Input  XmcBlockStatus=1  maskContainerNames=group1  block_type=slice  block_config=sysgen:Slice_config
  X : Outport
  Y : Outport  Port=2
  Z : Outport  Port=3
  wires:
  Slice/1 -> AddSub/3, AddSub2/3, Inverter/1
  Shift1/1 -> AddSub/2
  Shift/1 -> AddSub1/2
  Inverter/1 -> AddSub1/3
  Constant/1 -> AddSub2/2
  AddSub2/1 -> Z/1
  AddSub1/1 -> Y/1
  z/1 -> AddSub2/1
  AddSub/1 -> X/1
  y/1 -> Slice/1, Shift1/1, AddSub1/1
  x/1 -> Shift/1, AddSub/1

== system kay1024_freq_16ch_test/Subsystem/Subsystem16/Subsystem2/CORDIC ATAN/CORDIC Fine Angle PE/CORDIC PE8 ==
  note: X = x - y if y < 0, otherwise
      |    = x + y
      | Y = y + x if y < 0, otherwise
      |    = y - x
      | Z = z - atan(1/2^i) if y < 0, otherwise
      |    = z + atan(1/2^i)
  x : Inport
  y : Inport  Port=2
  z : Inport  Port=3
  AddSub : hdlBasic/AddSub  mode=Addition or Subtraction  use_carryin=off  use_carryout=off  en=off  latency=pipeline  precision=User Defined  arith_type="Signed  (2's comp)"  n_bits=pe_nbits  bin_pt=pe_binpt  quantization=Truncate  overflow=Wrap  use_behavioral_HDL=on  hw_selection=Fabric  pipelined=off  use_rpm=off  XmcBlockStatus=1  maskContainerNames=tabcontainer1  block_type=addsub  block_config=sysgen:Addsub_config
  AddSub1 : hdlBasic/AddSub  mode=Addition or Subtraction  use_carryin=off  use_carryout=off  en=off  latency=pipeline  precision=User Defined  arith_type="Signed  (2's comp)"  n_bits=pe_nbits  bin_pt=pe_binpt  quantization=Truncate  overflow=Wrap  use_behavioral_HDL=on  hw_selection=Fabric  pipelined=off  use_rpm=off  XmcBlockStatus=1  maskContainerNames=tabcontainer1  block_type=addsub  block_config=sysgen:Addsub_config
  AddSub2 : hdlBasic/AddSub  mode=Addition or Subtraction  use_carryin=off  use_carryout=off  en=off  latency=pipeline  precision=User Defined  arith_type="Signed  (2's comp)"  n_bits=pe_nbits  bin_pt=pe_binpt  quantization=Truncate  overflow=Wrap  use_behavioral_HDL=on  hw_selection=Fabric  pipelined=off  use_rpm=off  XmcBlockStatus=1  maskContainerNames=tabcontainer1  block_type=addsub  block_config=sysgen:Addsub_config
  Constant : hdlBasic/Constant  const=epsilon_k  gui_display_data_type=Fixed-point  arith_type=Signed (2's comp)  n_bits=pe_nbits  bin_pt=pe_binpt  preci_type=Single  exp_width=8  frac_width=24  explicit_period=off  period=1  XmcBlockStatus=1  maskContainerNames=tabcontainer1  block_type=constant  block_config=sysgen:Constant_config
  Inverter : hdlBasic/Inverter  en=off  latency=0  XmcBlockStatus=1  maskContainerNames=group2  block_type=inv  block_config=sysgen:Inverter_config
  Shift : hdlBasic/Shift  shift_dir=Right  shift_bits=ii  en=off  latency=0  precision=User Defined  arith_type="Signed  (2's comp)"  n_bits=pe_nbits  bin_pt=pe_binpt  quantization=Truncate  overflow=Wrap  XmcBlockStatus=1  maskContainerNames=group2  block_type=shift  block_config=sysgen:Shift_config
  Shift1 : hdlBasic/Shift  shift_dir=Right  shift_bits=ii  en=off  latency=0  precision=User Defined  arith_type="Signed  (2's comp)"  n_bits=pe_nbits  bin_pt=pe_binpt  quantization=Truncate  overflow=Wrap  XmcBlockStatus=1  maskContainerNames=group2  block_type=shift  block_config=sysgen:Shift_config
  Slice : hdlBasic/Slice  nbits=1  boolean_output=on  mode=Upper Bit Location + Width  bit1=0  base1=MSB of Input  bit0=0  base0=LSB of Input  XmcBlockStatus=1  maskContainerNames=group1  block_type=slice  block_config=sysgen:Slice_config
  X : Outport
  Y : Outport  Port=2
  Z : Outport  Port=3
  wires:
  Slice/1 -> AddSub/3, AddSub2/3, Inverter/1
  Shift1/1 -> AddSub/2
  Shift/1 -> AddSub1/2
  Inverter/1 -> AddSub1/3
  Constant/1 -> AddSub2/2
  AddSub2/1 -> Z/1
  AddSub1/1 -> Y/1
  z/1 -> AddSub2/1
  AddSub/1 -> X/1
  y/1 -> Slice/1, Shift1/1, AddSub1/1
  x/1 -> Shift/1, AddSub/1

== system kay1024_freq_16ch_test/Subsystem/Subsystem16/Subsystem2/CORDIC ATAN/CORDIC Fine Angle PE/CORDIC PE9 ==
  note: X = x - y if y < 0, otherwise
      |    = x + y
      | Y = y + x if y < 0, otherwise
      |    = y - x
      | Z = z - atan(1/2^i) if y < 0, otherwise
      |    = z + atan(1/2^i)
  x : Inport
  y : Inport  Port=2
  z : Inport  Port=3
  AddSub : hdlBasic/AddSub  mode=Addition or Subtraction  use_carryin=off  use_carryout=off  en=off  latency=pipeline  precision=User Defined  arith_type="Signed  (2's comp)"  n_bits=pe_nbits  bin_pt=pe_binpt  quantization=Truncate  overflow=Wrap  use_behavioral_HDL=on  hw_selection=Fabric  pipelined=off  use_rpm=off  XmcBlockStatus=1  maskContainerNames=tabcontainer1  block_type=addsub  block_config=sysgen:Addsub_config
  AddSub1 : hdlBasic/AddSub  mode=Addition or Subtraction  use_carryin=off  use_carryout=off  en=off  latency=pipeline  precision=User Defined  arith_type="Signed  (2's comp)"  n_bits=pe_nbits  bin_pt=pe_binpt  quantization=Truncate  overflow=Wrap  use_behavioral_HDL=on  hw_selection=Fabric  pipelined=off  use_rpm=off  XmcBlockStatus=1  maskContainerNames=tabcontainer1  block_type=addsub  block_config=sysgen:Addsub_config
  AddSub2 : hdlBasic/AddSub  mode=Addition or Subtraction  use_carryin=off  use_carryout=off  en=off  latency=pipeline  precision=User Defined  arith_type="Signed  (2's comp)"  n_bits=pe_nbits  bin_pt=pe_binpt  quantization=Truncate  overflow=Wrap  use_behavioral_HDL=on  hw_selection=Fabric  pipelined=off  use_rpm=off  XmcBlockStatus=1  maskContainerNames=tabcontainer1  block_type=addsub  block_config=sysgen:Addsub_config
  Constant : hdlBasic/Constant  const=epsilon_k  gui_display_data_type=Fixed-point  arith_type=Signed (2's comp)  n_bits=pe_nbits  bin_pt=pe_binpt  preci_type=Single  exp_width=8  frac_width=24  explicit_period=off  period=1  XmcBlockStatus=1  maskContainerNames=tabcontainer1  block_type=constant  block_config=sysgen:Constant_config
  Inverter : hdlBasic/Inverter  en=off  latency=0  XmcBlockStatus=1  maskContainerNames=group2  block_type=inv  block_config=sysgen:Inverter_config
  Shift : hdlBasic/Shift  shift_dir=Right  shift_bits=ii  en=off  latency=0  precision=User Defined  arith_type="Signed  (2's comp)"  n_bits=pe_nbits  bin_pt=pe_binpt  quantization=Truncate  overflow=Wrap  XmcBlockStatus=1  maskContainerNames=group2  block_type=shift  block_config=sysgen:Shift_config
  Shift1 : hdlBasic/Shift  shift_dir=Right  shift_bits=ii  en=off  latency=0  precision=User Defined  arith_type="Signed  (2's comp)"  n_bits=pe_nbits  bin_pt=pe_binpt  quantization=Truncate  overflow=Wrap  XmcBlockStatus=1  maskContainerNames=group2  block_type=shift  block_config=sysgen:Shift_config
  Slice : hdlBasic/Slice  nbits=1  boolean_output=on  mode=Upper Bit Location + Width  bit1=0  base1=MSB of Input  bit0=0  base0=LSB of Input  XmcBlockStatus=1  maskContainerNames=group1  block_type=slice  block_config=sysgen:Slice_config
  X : Outport
  Y : Outport  Port=2
  Z : Outport  Port=3
  wires:
  Slice/1 -> AddSub/3, AddSub2/3, Inverter/1
  Shift1/1 -> AddSub/2
  Shift/1 -> AddSub1/2
  Inverter/1 -> AddSub1/3
  Constant/1 -> AddSub2/2
  AddSub2/1 -> Z/1
  AddSub1/1 -> Y/1
  z/1 -> AddSub2/1
  AddSub/1 -> X/1
  y/1 -> Slice/1, Shift1/1, AddSub1/1
  x/1 -> Shift/1, AddSub/1

== system kay1024_freq_16ch_test/Subsystem/Subsystem16/Subsystem3/CORDIC ATAN/CORDIC Fine Angle PE/CORDIC PE1 ==
  note: X = x - y if y < 0, otherwise
      |    = x + y
      | Y = y + x if y < 0, otherwise
      |    = y - x
      | Z = z - atan(1/2^i) if y < 0, otherwise
      |    = z + atan(1/2^i)
  x : Inport
  y : Inport  Port=2
  z : Inport  Port=3
  AddSub : hdlBasic/AddSub  mode=Addition or Subtraction  use_carryin=off  use_carryout=off  en=off  latency=pipeline  precision=User Defined  arith_type="Signed  (2's comp)"  n_bits=pe_nbits  bin_pt=pe_binpt  quantization=Truncate  overflow=Wrap  use_behavioral_HDL=on  hw_selection=Fabric  pipelined=off  use_rpm=off  XmcBlockStatus=1  maskContainerNames=tabcontainer1  block_type=addsub  block_config=sysgen:Addsub_config
  AddSub1 : hdlBasic/AddSub  mode=Addition or Subtraction  use_carryin=off  use_carryout=off  en=off  latency=pipeline  precision=User Defined  arith_type="Signed  (2's comp)"  n_bits=pe_nbits  bin_pt=pe_binpt  quantization=Truncate  overflow=Wrap  use_behavioral_HDL=on  hw_selection=Fabric  pipelined=off  use_rpm=off  XmcBlockStatus=1  maskContainerNames=tabcontainer1  block_type=addsub  block_config=sysgen:Addsub_config
  AddSub2 : hdlBasic/AddSub  mode=Addition or Subtraction  use_carryin=off  use_carryout=off  en=off  latency=pipeline  precision=User Defined  arith_type="Signed  (2's comp)"  n_bits=pe_nbits  bin_pt=pe_binpt  quantization=Truncate  overflow=Wrap  use_behavioral_HDL=on  hw_selection=Fabric  pipelined=off  use_rpm=off  XmcBlockStatus=1  maskContainerNames=tabcontainer1  block_type=addsub  block_config=sysgen:Addsub_config
  Constant : hdlBasic/Constant  const=epsilon_k  gui_display_data_type=Fixed-point  arith_type=Signed (2's comp)  n_bits=pe_nbits  bin_pt=pe_binpt  preci_type=Single  exp_width=8  frac_width=24  explicit_period=off  period=1  XmcBlockStatus=1  maskContainerNames=tabcontainer1  block_type=constant  block_config=sysgen:Constant_config
  Inverter : hdlBasic/Inverter  en=off  latency=0  XmcBlockStatus=1  maskContainerNames=group2  block_type=inv  block_config=sysgen:Inverter_config
  Shift : hdlBasic/Shift  shift_dir=Right  shift_bits=ii  en=off  latency=0  precision=User Defined  arith_type="Signed  (2's comp)"  n_bits=pe_nbits  bin_pt=pe_binpt  quantization=Truncate  overflow=Wrap  XmcBlockStatus=1  maskContainerNames=group2  block_type=shift  block_config=sysgen:Shift_config
  Shift1 : hdlBasic/Shift  shift_dir=Right  shift_bits=ii  en=off  latency=0  precision=User Defined  arith_type="Signed  (2's comp)"  n_bits=pe_nbits  bin_pt=pe_binpt  quantization=Truncate  overflow=Wrap  XmcBlockStatus=1  maskContainerNames=group2  block_type=shift  block_config=sysgen:Shift_config
  Slice : hdlBasic/Slice  nbits=1  boolean_output=on  mode=Upper Bit Location + Width  bit1=0  base1=MSB of Input  bit0=0  base0=LSB of Input  XmcBlockStatus=1  maskContainerNames=group1  block_type=slice  block_config=sysgen:Slice_config
  X : Outport
  Y : Outport  Port=2
  Z : Outport  Port=3
  wires:
  x/1 -> AddSub/1, Shift/1
  y/1 -> AddSub1/1, Shift1/1, Slice/1
  AddSub/1 -> X/1
  z/1 -> AddSub2/1
  AddSub1/1 -> Y/1
  AddSub2/1 -> Z/1
  Constant/1 -> AddSub2/2
  Inverter/1 -> AddSub1/3
  Shift/1 -> AddSub1/2
  Shift1/1 -> AddSub/2
  Slice/1 -> Inverter/1, AddSub2/3, AddSub/3

== system kay1024_freq_16ch_test/Subsystem/Subsystem16/Subsystem3/CORDIC ATAN/CORDIC Fine Angle PE/CORDIC PE10 ==
  note: X = x - y if y < 0, otherwise
      |    = x + y
      | Y = y + x if y < 0, otherwise
      |    = y - x
      | Z = z - atan(1/2^i) if y < 0, otherwise
      |    = z + atan(1/2^i)
  x : Inport
  y : Inport  Port=2
  z : Inport  Port=3
  AddSub : hdlBasic/AddSub  mode=Addition or Subtraction  use_carryin=off  use_carryout=off  en=off  latency=pipeline  precision=User Defined  arith_type="Signed  (2's comp)"  n_bits=pe_nbits  bin_pt=pe_binpt  quantization=Truncate  overflow=Wrap  use_behavioral_HDL=on  hw_selection=Fabric  pipelined=off  use_rpm=off  XmcBlockStatus=1  maskContainerNames=tabcontainer1  block_type=addsub  block_config=sysgen:Addsub_config
  AddSub1 : hdlBasic/AddSub  mode=Addition or Subtraction  use_carryin=off  use_carryout=off  en=off  latency=pipeline  precision=User Defined  arith_type="Signed  (2's comp)"  n_bits=pe_nbits  bin_pt=pe_binpt  quantization=Truncate  overflow=Wrap  use_behavioral_HDL=on  hw_selection=Fabric  pipelined=off  use_rpm=off  XmcBlockStatus=1  maskContainerNames=tabcontainer1  block_type=addsub  block_config=sysgen:Addsub_config
  AddSub2 : hdlBasic/AddSub  mode=Addition or Subtraction  use_carryin=off  use_carryout=off  en=off  latency=pipeline  precision=User Defined  arith_type="Signed  (2's comp)"  n_bits=pe_nbits  bin_pt=pe_binpt  quantization=Truncate  overflow=Wrap  use_behavioral_HDL=on  hw_selection=Fabric  pipelined=off  use_rpm=off  XmcBlockStatus=1  maskContainerNames=tabcontainer1  block_type=addsub  block_config=sysgen:Addsub_config
  Constant : hdlBasic/Constant  const=epsilon_k  gui_display_data_type=Fixed-point  arith_type=Signed (2's comp)  n_bits=pe_nbits  bin_pt=pe_binpt  preci_type=Single  exp_width=8  frac_width=24  explicit_period=off  period=1  XmcBlockStatus=1  maskContainerNames=tabcontainer1  block_type=constant  block_config=sysgen:Constant_config
  Inverter : hdlBasic/Inverter  en=off  latency=0  XmcBlockStatus=1  maskContainerNames=group2  block_type=inv  block_config=sysgen:Inverter_config
  Shift : hdlBasic/Shift  shift_dir=Right  shift_bits=ii  en=off  latency=0  precision=User Defined  arith_type="Signed  (2's comp)"  n_bits=pe_nbits  bin_pt=pe_binpt  quantization=Truncate  overflow=Wrap  XmcBlockStatus=1  maskContainerNames=group2  block_type=shift  block_config=sysgen:Shift_config
  Shift1 : hdlBasic/Shift  shift_dir=Right  shift_bits=ii  en=off  latency=0  precision=User Defined  arith_type="Signed  (2's comp)"  n_bits=pe_nbits  bin_pt=pe_binpt  quantization=Truncate  overflow=Wrap  XmcBlockStatus=1  maskContainerNames=group2  block_type=shift  block_config=sysgen:Shift_config
  Slice : hdlBasic/Slice  nbits=1  boolean_output=on  mode=Upper Bit Location + Width  bit1=0  base1=MSB of Input  bit0=0  base0=LSB of Input  XmcBlockStatus=1  maskContainerNames=group1  block_type=slice  block_config=sysgen:Slice_config
  X : Outport
  Y : Outport  Port=2
  Z : Outport  Port=3
  wires:
  Slice/1 -> AddSub/3, AddSub2/3, Inverter/1
  Shift1/1 -> AddSub/2
  Shift/1 -> AddSub1/2
  Inverter/1 -> AddSub1/3
  Constant/1 -> AddSub2/2
  AddSub2/1 -> Z/1
  AddSub1/1 -> Y/1
  z/1 -> AddSub2/1
  AddSub/1 -> X/1
  y/1 -> Slice/1, Shift1/1, AddSub1/1
  x/1 -> Shift/1, AddSub/1
